simulink model "DCX_CHW_Hydraulics_SSC"  (R2024a)
settings: Solver=ode23t  StartTime=0.0  StopTime=30  MaxStep=0.5  RelTol=1e-3
values from neighbouring files (symbols this model uses):
  P = dcx_params('Profile', opts.Profile); assignin('base', 'P', P)    [dcx_validate_hydraulics.m]
undefined symbols (not defined in the file or in its folder): ssc_iso, ssc_n, ssc_v
libraries: fl_lib x29, nesl_utility x13, SimscapeFluids_lib x2
settings Model: Creator=deshm  LastModifiedBy=deshm
settings DataIOCC: SaveFormat=Array

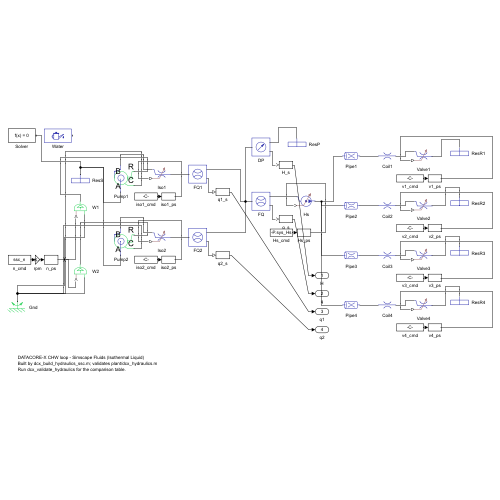
[thumbnail: Simulink's stored preview of the top-level diagram]
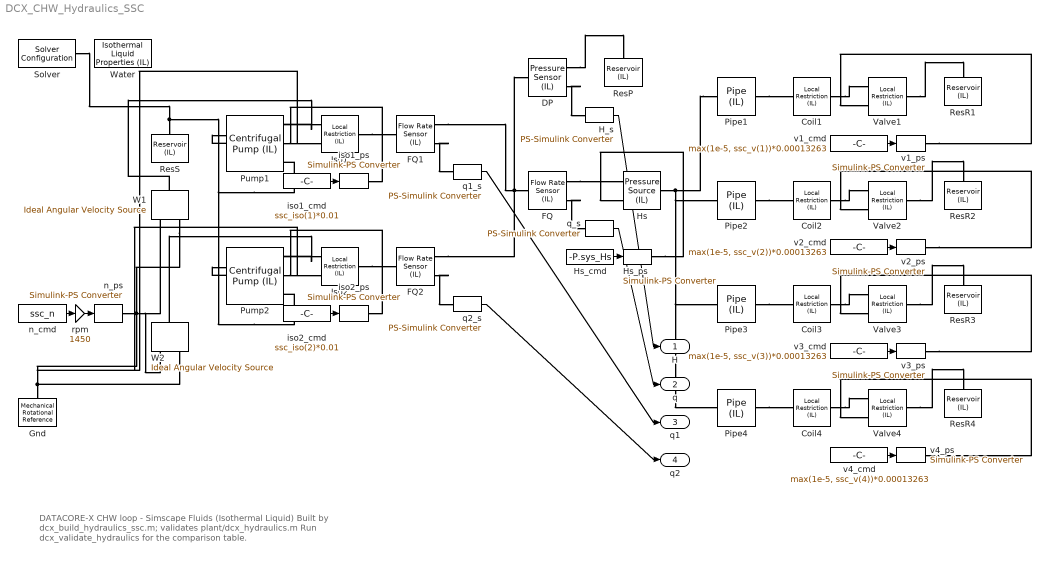
== system DCX_CHW_Hydraulics_SSC ==
  note: DATACORE-X CHW loop - Simscape Fluids (Isothermal Liquid)
      | Built by dcx_build_hydraulics_ssc.m; validates plant/dcx_hydraulics.m
      | Run dcx_validate_hydraulics for the comparison table.
  Coil{1..4} (4 alike) : fl_lib/Isothermal Liquid/Elements/Local Restriction (IL)  restriction_type=foundation.enum.restriction_type.fixed  restriction_area=0.000255 m^2  min_area=1e-10 m^2  max_area=0.005 m^2  area=inf m^2  Cd=0.64  Re_c=150  pressure_recovery=false
      settings: InternalSimscapePortConfiguration="{\"Bottom\":[],\"Left\":[{\"id\":\"A\",\"label\":\"A\",\"type\":\"foundation.isothermal_liquid.isothermal_liquid\"}],\"Right\":[{\"id\":\"B\",\"label\":\"B\",\"type\":\"foundation.isothermal_liquid.isothermal_liquid\"}],\"Top\":[]}"
  DP : fl_lib/Isothermal Liquid/Sensors/Pressure Sensor (IL)  pressure_measure=foundation.enum.pressure_measure.difference
      settings: InternalSimscapePortConfiguration="{\"Bottom\":[],\"Left\":[{\"id\":\"A\",\"label\":\"A\",\"type\":\"foundation.isothermal_liquid.isothermal_liquid\"}],\"Right\":[{\"id\":\"B\",\"label\":\"B\",\"type\":\"foundation.isothermal_liquid.isothermal_liquid\"},{\"id\":\"P\",\"label\":\"P\",\"type\":\"output\"}],\"Top\":[]}"
  FQ : fl_lib/Isothermal Liquid/Sensors/Flow Rate Sensor (IL)  sensor_type=foundation.enum.mass_volumetric_sensor.mass
      settings: InternalSimscapePortConfiguration="{\"Bottom\":[],\"Left\":[{\"id\":\"A\",\"label\":\"A\",\"type\":\"foundation.isothermal_liquid.isothermal_liquid\"}],\"Right\":[{\"id\":\"B\",\"label\":\"B\",\"type\":\"foundation.isothermal_liquid.isothermal_liquid\"},{\"id\":\"M\",\"label\":\"M\",\"type\":\"output\"}],\"Top\":[]}"
  FQ1 : fl_lib/Isothermal Liquid/Sensors/Flow Rate Sensor (IL)  sensor_type=foundation.enum.mass_volumetric_sensor.mass
      settings: InternalSimscapePortConfiguration="{\"Bottom\":[],\"Left\":[{\"id\":\"A\",\"label\":\"A\",\"type\":\"foundation.isothermal_liquid.isothermal_liquid\"}],\"Right\":[{\"id\":\"B\",\"label\":\"B\",\"type\":\"foundation.isothermal_liquid.isothermal_liquid\"},{\"id\":\"M\",\"label\":\"M\",\"type\":\"output\"}],\"Top\":[]}"
  FQ2 : fl_lib/Isothermal Liquid/Sensors/Flow Rate Sensor (IL)  sensor_type=foundation.enum.mass_volumetric_sensor.mass
      settings: InternalSimscapePortConfiguration="{\"Bottom\":[],\"Left\":[{\"id\":\"A\",\"label\":\"A\",\"type\":\"foundation.isothermal_liquid.isothermal_liquid\"}],\"Right\":[{\"id\":\"B\",\"label\":\"B\",\"type\":\"foundation.isothermal_liquid.isothermal_liquid\"},{\"id\":\"M\",\"label\":\"M\",\"type\":\"output\"}],\"Top\":[]}"
  Gnd : fl_lib/Mechanical/Rotational Elements/Mechanical Rotational Reference
  H_s : nesl_utility/PS-Simulink Converter  PhysicalDomain=network_engine_domain  SubClassName=ps_output  LeftPortType=input  RightPortType=output  PseudoPeriodic=off  Frequencies=[]  VectorFormat=inherit  Unit=kPa  AffineConversion=off
  Hs : fl_lib/Isothermal Liquid/Sources/Pressure Source (IL)  source_type=foundation.enum.constant_controlled.controlled  pressure_differential=0 MPa
      settings: InternalSimscapePortConfiguration="{\"Bottom\":[],\"Left\":[{\"id\":\"A\",\"label\":\"A\",\"type\":\"foundation.isothermal_liquid.isothermal_liquid\"},{\"id\":\"P\",\"label\":\"P\",\"type\":\"input\"}],\"Right\":[{\"id\":\"B\",\"label\":\"B\",\"type\":\"foundation.isothermal_liquid.isothermal_liquid\"}],\"Top\":[]}"
  Hs_cmd : Constant  Value=-P.sys_Hs
  Hs_ps : nesl_utility/Simulink-PS Converter  PhysicalDomain=network_engine_domain  SubClassName=ps_input  LeftPortType=input  RightPortType=output  PseudoPeriodic=off  Frequencies=[]  NoiseDistribution=none  NoiseParameters=[]  Unit=kPa  AffineConversion=off  FilteringAndDerivatives=provide  SimscapeFilterOrder=1  InputFilterTimeConstant=0.001  UdotUserProvided=0
  Iso1 : fl_lib/Isothermal Liquid/Elements/Local Restriction (IL)  restriction_type=foundation.enum.restriction_type.variable  restriction_area=1e-3 m^2  min_area=1e-9 m^2  max_area=0.01 m^2  area=inf m^2  Cd=0.9  Re_c=150  pressure_recovery=false
      settings: InternalSimscapePortConfiguration="{\"Bottom\":[],\"Left\":[{\"id\":\"A\",\"label\":\"A\",\"type\":\"foundation.isothermal_liquid.isothermal_liquid\"},{\"id\":\"AR\",\"label\":\"AR\",\"type\":\"input\"}],\"Right\":[{\"id\":\"B\",\"label\":\"B\",\"type\":\"foundation.isothermal_liquid.isothermal_liquid\"}],\"Top\":[]}"
  Iso2 : fl_lib/Isothermal Liquid/Elements/Local Restriction (IL)  restriction_type=foundation.enum.restriction_type.variable  restriction_area=1e-3 m^2  min_area=1e-9 m^2  max_area=0.01 m^2  area=inf m^2  Cd=0.9  Re_c=150  pressure_recovery=false
      settings: InternalSimscapePortConfiguration="{\"Bottom\":[],\"Left\":[{\"id\":\"A\",\"label\":\"A\",\"type\":\"foundation.isothermal_liquid.isothermal_liquid\"},{\"id\":\"AR\",\"label\":\"AR\",\"type\":\"input\"}],\"Right\":[{\"id\":\"B\",\"label\":\"B\",\"type\":\"foundation.isothermal_liquid.isothermal_liquid\"}],\"Top\":[]}"
  Pipe{1..4} (4 alike) : fl_lib/Isothermal Liquid/Elements/Pipe (IL)  length=40 m  area=0.0013203 m^2  Dh=0.041 m  length_add=6 m  roughness=15e-6 m  Re_lam=2000  Re_tur=4000  shape_factor=64  dynamic_compressibility=true  inertia=false  p0=0.6 MPa  mdot0=0 kg/s
      settings: InternalSimscapePortConfiguration="{\"Bottom\":[],\"Left\":[{\"id\":\"A\",\"label\":\"A\",\"type\":\"foundation.isothermal_liquid.isothermal_liquid\"}],\"Right\":[{\"id\":\"B\",\"label\":\"B\",\"type\":\"foundation.isothermal_liquid.isothermal_liquid\"}],\"Top\":[]}"
  Pump1 : SimscapeFluids_lib/Isothermal Liquid/Pumps & Motors/Centrifugal Pump (IL)  pump_parameterization=fluids.isothermal_liquid.pumps_motors.enum.centrifugal_pump_spec.table1D  capacity_ref_nominal=45 lpm  head_ref_nominal=40 m  power_ref_nominal=0.85 kW  head_ref_max=60 m  capacity_ref_max=80 lpm  omega_ref_analytic=1770 rpm  capacity_ref_1D_TLU=[0 0.00106351 0.00212703 0.00319054 0.00425405 0.00531756 0.00638108 0.00744459 0.0085081 0.00957161 0.0106351 0.0116986] m^3/s  head_ref_1D_TLU=[32.6894 32.4352 31.6727 30.4017 28.6223 26.3346 23.5384 20.2339 16.421 12.0997 7.27002 1.93195] m  power_ref_1D_TLU=[0.2 0.930309 1.2447 1.47312 1.68547 1.91009 2.17487 2.53225 3.13357 4.75407 5.0458 1.47496] kW  omega_ref_1D=1450 rpm  rho_ref_1D=998.21 kg/m^3  omega_threshold_factor=1e-2  capacity_2D_TLU=[16.67, 23.33, 30, 40, 53.33, 60] lpm  omega_2D_TLU=[2450, 2800, 3150, 3500] rpm  head_2D_TLU=[25, 32.7, 42.5, 50; 24, 31.7, 41, 49; 22.7, 30.5, 39, 47.5; 20, 28, 36, 45; 15.7, 24, 32, 40; 12.5, 21, 29.5, 37.5] m  power_2D_TLU=[.28, .38, .5, .6; .31, .41, .55, .68; .33, .44, .6, .75; .36, .48, .65, .83; .38, .53, .72, .93; .39, .55, .75, .97] kW  rho_ref_2D=998.21 kg/m^3  diameter_ratio=1  mech_orientation=fluids.isothermal_liquid.pumps_motors.enum.centrifugal_pump_mech_orientation.positive  operation_check=simscape.enum.assert.action.none
      settings: InternalSimscapePortConfiguration="{\"Bottom\":[{\"id\":\"A\",\"label\":\"A\",\"type\":\"foundation.isothermal_liquid.isothermal_liquid\"}],\"Left\":[],\"Right\":[{\"id\":\"R\",\"label\":\"R\",\"type\":\"foundation.mechanical.rotational.rotational\"},{\"id\":\"C\",\"label\":\"C\",\"type\":\"foundation.mechanical.rotational.rotational\"}],\"Top\":[{\"id\":\"B\",\"label\":\"B\",\"type\":\"foundation.isothermal_liquid.isothermal_liquid\"}]}"
  Pump2 : SimscapeFluids_lib/Isothermal Liquid/Pumps & Motors/Centrifugal Pump (IL)  pump_parameterization=fluids.isothermal_liquid.pumps_motors.enum.centrifugal_pump_spec.table1D  capacity_ref_nominal=45 lpm  head_ref_nominal=40 m  power_ref_nominal=0.85 kW  head_ref_max=60 m  capacity_ref_max=80 lpm  omega_ref_analytic=1770 rpm  capacity_ref_1D_TLU=[0 0.00106351 0.00212703 0.00319054 0.00425405 0.00531756 0.00638108 0.00744459 0.0085081 0.00957161 0.0106351 0.0116986] m^3/s  head_ref_1D_TLU=[32.6894 32.4352 31.6727 30.4017 28.6223 26.3346 23.5384 20.2339 16.421 12.0997 7.27002 1.93195] m  power_ref_1D_TLU=[0.2 0.930309 1.2447 1.47312 1.68547 1.91009 2.17487 2.53225 3.13357 4.75407 5.0458 1.47496] kW  omega_ref_1D=1450 rpm  rho_ref_1D=998.21 kg/m^3  omega_threshold_factor=1e-2  capacity_2D_TLU=[16.67, 23.33, 30, 40, 53.33, 60] lpm  omega_2D_TLU=[2450, 2800, 3150, 3500] rpm  head_2D_TLU=[25, 32.7, 42.5, 50; 24, 31.7, 41, 49; 22.7, 30.5, 39, 47.5; 20, 28, 36, 45; 15.7, 24, 32, 40; 12.5, 21, 29.5, 37.5] m  power_2D_TLU=[.28, .38, .5, .6; .31, .41, .55, .68; .33, .44, .6, .75; .36, .48, .65, .83; .38, .53, .72, .93; .39, .55, .75, .97] kW  rho_ref_2D=998.21 kg/m^3  diameter_ratio=1  mech_orientation=fluids.isothermal_liquid.pumps_motors.enum.centrifugal_pump_mech_orientation.positive  operation_check=simscape.enum.assert.action.none
      settings: InternalSimscapePortConfiguration="{\"Bottom\":[{\"id\":\"A\",\"label\":\"A\",\"type\":\"foundation.isothermal_liquid.isothermal_liquid\"}],\"Left\":[],\"Right\":[{\"id\":\"R\",\"label\":\"R\",\"type\":\"foundation.mechanical.rotational.rotational\"},{\"id\":\"C\",\"label\":\"C\",\"type\":\"foundation.mechanical.rotational.rotational\"}],\"Top\":[{\"id\":\"B\",\"label\":\"B\",\"type\":\"foundation.isothermal_liquid.isothermal_liquid\"}]}"
  ResP : fl_lib/Isothermal Liquid/Elements/Reservoir (IL)  reservoir_type=foundation.enum.constant_controlled.constant  pressure_spec=foundation.enum.pressure_spec.specified  reservoir_pressure=0.6 MPa
  ResR{1..4} (4 alike) : fl_lib/Isothermal Liquid/Elements/Reservoir (IL)  reservoir_type=foundation.enum.constant_controlled.constant  pressure_spec=foundation.enum.pressure_spec.specified  reservoir_pressure=0.6 MPa
  ResS : fl_lib/Isothermal Liquid/Elements/Reservoir (IL)  reservoir_type=foundation.enum.constant_controlled.constant  pressure_spec=foundation.enum.pressure_spec.specified  reservoir_pressure=0.6 MPa
  Solver : nesl_utility/Solver Configuration  PhysicalDomain=network_engine_domain  SubClassName=solver  LeftPortType=input  RightPortType=generic  Tones=[]  Harmonics=[]  SimulateNoise=off  Profile=off  UseLocalSampling=off  EnableSwitchedLinearOptims=on  FrequencyDomain=off  UseCCode=off  RelTol=0.001  AbsTol=0.001  MinStep=1e-09  ToWorkspace=off  RevertToSquareIcSolve=off  NumHomotopyIterations=100  PhasorMode=off  PhasorModeNumHarmonics=1  ConsistencySolver=NEWTON_XTOL_AFTER_FTOL  IndexReductionMethod=DerivativeReplacement  DoDC=off  ResidualTolerance=1e-09  ConsistencyTolSource=GLOBAL  ConsistencyAbsTol=0.001  ConsistencyRelTol=0.001  ConsistencyTolFactor=0.001  UseLocalSolver=off  LocalSolverChoice=NE_BACKWARD_EULER_ADVANCER  ResolveIndetEquations=on  FunctionEvalNumThread=1  LocalSolverSampleTime=0.001  DoFixedCost=off  MaxNonlinIter=3  MaxModeIter=2  ComputeImpulses=off  ImpulseIterations=2  LinearAlgebra=auto  LinearAlgebraNumThread=0  EquationFormulation=NE_TIME_EF  DelaysMemoryBudget=1024  AutomaticFiltering=on  FilteringTimeConstant=0.001  PartitionStorageMethod=AS_NEEDED  PartitionMemoryBudget=1024  PartitionMethod=ROBUST  MultibodyUseLocalSolver=off  MultibodyLocalSolverChoice=ODE1  MultibodyLocalSolverSampleTime=0.001
  Valve{1..4} (4 alike) : fl_lib/Isothermal Liquid/Elements/Local Restriction (IL)  restriction_type=foundation.enum.restriction_type.variable  restriction_area=1e-3 m^2  min_area=1e-9 m^2  max_area=0.00013263 m^2  area=inf m^2  Cd=0.64  Re_c=150  pressure_recovery=false
      settings: InternalSimscapePortConfiguration="{\"Bottom\":[],\"Left\":[{\"id\":\"A\",\"label\":\"A\",\"type\":\"foundation.isothermal_liquid.isothermal_liquid\"},{\"id\":\"AR\",\"label\":\"AR\",\"type\":\"input\"}],\"Right\":[{\"id\":\"B\",\"label\":\"B\",\"type\":\"foundation.isothermal_liquid.isothermal_liquid\"}],\"Top\":[]}"
  W1 : fl_lib/Mechanical/Mechanical Sources/Ideal Angular Velocity Source
  W2 : fl_lib/Mechanical/Mechanical Sources/Ideal Angular Velocity Source
  Water : fl_lib/Isothermal Liquid/Utilities/Isothermal Liquid Properties (IL)  rho_L_atm=998.21 kg/m^3  bulk_modulus_model=foundation.enum.bulk_modulus_model.const  beta_gain=6  beta_L_atm=2.1791e9 Pa  nu_atm=1.0034e-6 m^2/s  p_atm=0.101325 MPa  p_min=1 Pa  properties_range_check=simscape.enum.assert.action.error  air_fraction=0.005  polytropic_index=1.0  rho_g_atm=1.225 kg/m^3  air_dissolution_model=false  p_crit=3 MPa
  iso1_cmd : Constant  Value=ssc_iso(1)*0.01
  iso1_ps : nesl_utility/Simulink-PS Converter  PhysicalDomain=network_engine_domain  SubClassName=ps_input  LeftPortType=input  RightPortType=output  PseudoPeriodic=off  Frequencies=[]  NoiseDistribution=none  NoiseParameters=[]  Unit=m^2  AffineConversion=off  FilteringAndDerivatives=provide  SimscapeFilterOrder=1  InputFilterTimeConstant=0.001  UdotUserProvided=0
  iso2_cmd : Constant  Value=ssc_iso(2)*0.01
  iso2_ps : nesl_utility/Simulink-PS Converter  PhysicalDomain=network_engine_domain  SubClassName=ps_input  LeftPortType=input  RightPortType=output  PseudoPeriodic=off  Frequencies=[]  NoiseDistribution=none  NoiseParameters=[]  Unit=m^2  AffineConversion=off  FilteringAndDerivatives=provide  SimscapeFilterOrder=1  InputFilterTimeConstant=0.001  UdotUserProvided=0
  n_cmd : Constant  Value=ssc_n
  n_ps : nesl_utility/Simulink-PS Converter  PhysicalDomain=network_engine_domain  SubClassName=ps_input  LeftPortType=input  RightPortType=output  PseudoPeriodic=off  Frequencies=[]  NoiseDistribution=none  NoiseParameters=[]  Unit=rpm  AffineConversion=off  FilteringAndDerivatives=provide  SimscapeFilterOrder=1  InputFilterTimeConstant=0.001  UdotUserProvided=0
  q1_s : nesl_utility/PS-Simulink Converter  PhysicalDomain=network_engine_domain  SubClassName=ps_output  LeftPortType=input  RightPortType=output  PseudoPeriodic=off  Frequencies=[]  VectorFormat=inherit  Unit=kg/s  AffineConversion=off
  q2_s : nesl_utility/PS-Simulink Converter  PhysicalDomain=network_engine_domain  SubClassName=ps_output  LeftPortType=input  RightPortType=output  PseudoPeriodic=off  Frequencies=[]  VectorFormat=inherit  Unit=kg/s  AffineConversion=off
  q_s : nesl_utility/PS-Simulink Converter  PhysicalDomain=network_engine_domain  SubClassName=ps_output  LeftPortType=input  RightPortType=output  PseudoPeriodic=off  Frequencies=[]  VectorFormat=inherit  Unit=kg/s  AffineConversion=off
  rpm : Gain  Gain=1450
  v1_cmd : Constant  Value=max(1e-5, ssc_v(1))*0.00013263
  v1_ps : nesl_utility/Simulink-PS Converter  PhysicalDomain=network_engine_domain  SubClassName=ps_input  LeftPortType=input  RightPortType=output  PseudoPeriodic=off  Frequencies=[]  NoiseDistribution=none  NoiseParameters=[]  Unit=m^2  AffineConversion=off  FilteringAndDerivatives=provide  SimscapeFilterOrder=1  InputFilterTimeConstant=0.001  UdotUserProvided=0
  v2_cmd : Constant  Value=max(1e-5, ssc_v(2))*0.00013263
  v2_ps : nesl_utility/Simulink-PS Converter  PhysicalDomain=network_engine_domain  SubClassName=ps_input  LeftPortType=input  RightPortType=output  PseudoPeriodic=off  Frequencies=[]  NoiseDistribution=none  NoiseParameters=[]  Unit=m^2  AffineConversion=off  FilteringAndDerivatives=provide  SimscapeFilterOrder=1  InputFilterTimeConstant=0.001  UdotUserProvided=0
  v3_cmd : Constant  Value=max(1e-5, ssc_v(3))*0.00013263
  v3_ps : nesl_utility/Simulink-PS Converter  PhysicalDomain=network_engine_domain  SubClassName=ps_input  LeftPortType=input  RightPortType=output  PseudoPeriodic=off  Frequencies=[]  NoiseDistribution=none  NoiseParameters=[]  Unit=m^2  AffineConversion=off  FilteringAndDerivatives=provide  SimscapeFilterOrder=1  InputFilterTimeConstant=0.001  UdotUserProvided=0
  v4_cmd : Constant  Value=max(1e-5, ssc_v(4))*0.00013263
  v4_ps : nesl_utility/Simulink-PS Converter  PhysicalDomain=network_engine_domain  SubClassName=ps_input  LeftPortType=input  RightPortType=output  PseudoPeriodic=off  Frequencies=[]  NoiseDistribution=none  NoiseParameters=[]  Unit=m^2  AffineConversion=off  FilteringAndDerivatives=provide  SimscapeFilterOrder=1  InputFilterTimeConstant=0.001  UdotUserProvided=0
  H : Outport
  q : Outport  Port=2
  q1 : Outport  Port=3
  q2 : Outport  Port=4
  wires:
  n_cmd/1 -> rpm/1
  rpm/1 -> n_ps/1
  iso1_cmd/1 -> iso1_ps/1
  iso2_cmd/1 -> iso2_ps/1
  Hs_cmd/1 -> Hs_ps/1
  v1_cmd/1 -> v1_ps/1
  v2_cmd/1 -> v2_ps/1
  v3_cmd/1 -> v3_ps/1
  v4_cmd/1 -> v4_ps/1
  H_s/1 -> H/1
  q_s/1 -> q/1
  q1_s/1 -> q1/1
  q2_s/1 -> q2/1
  connections:
  Solver/RConn1 -- Pump1/RConn3 -- ResS/LConn1 -- Pump2/RConn3
  Pump1/LConn1 -- Iso1/LConn1
  W1/RConn1 -- n_ps/RConn1 -- W2/RConn1
  W1/LConn1 -- Pump1/RConn1
  W1/RConn2 -- Pump1/RConn2 -- W2/RConn2 -- Gnd/LConn1 -- Pump2/RConn2
  iso1_ps/RConn1 -- Iso1/LConn2
  Iso1/RConn1 -- FQ1/LConn1
  FQ1/RConn1 -- FQ2/RConn1 -- FQ/LConn1 -- DP/LConn1
  FQ1/RConn2 -- q1_s/LConn1
  Pump2/LConn1 -- Iso2/LConn1
  W2/LConn1 -- Pump2/RConn1
  iso2_ps/RConn1 -- Iso2/LConn2
  Iso2/RConn1 -- FQ2/LConn1
  FQ2/RConn2 -- q2_s/LConn1
  DP/RConn1 -- ResP/LConn1
  DP/RConn2 -- H_s/LConn1
  FQ/RConn2 -- q_s/LConn1
  FQ/RConn1 -- Hs/LConn1
  Hs_ps/RConn1 -- Hs/LConn2
  Pipe1/LConn1 -- Hs/RConn1 -- Pipe2/LConn1 -- Pipe3/LConn1 -- Pipe4/LConn1
  Pipe1/RConn1 -- Coil1/LConn1
  Coil1/RConn1 -- Valve1/LConn1
  v1_ps/RConn1 -- Valve1/LConn2
  Valve1/RConn1 -- ResR1/LConn1
  Pipe2/RConn1 -- Coil2/LConn1
  Coil2/RConn1 -- Valve2/LConn1
  v2_ps/RConn1 -- Valve2/LConn2
  Valve2/RConn1 -- ResR2/LConn1
  Pipe3/RConn1 -- Coil3/LConn1
  Coil3/RConn1 -- Valve3/LConn1
  v3_ps/RConn1 -- Valve3/LConn2
  Valve3/RConn1 -- ResR3/LConn1
  Pipe4/RConn1 -- Coil4/LConn1
  Coil4/RConn1 -- Valve4/LConn1
  v4_ps/RConn1 -- Valve4/LConn2
  Valve4/RConn1 -- ResR4/LConn1
